simulink model "Inverse_Clark_Park_Transform"  (R2021a)
settings: Solver=FixedStepAuto  StartTime=0.0  StopTime=10  FixedStep=2e-5  RelTol=1e-6
InitFcn:
  | cd 'F:\Learning\Power\FOC';
  | run('Params.m')
settings Model: Creator=DEEL  LastModifiedBy=DEEL
settings SolverCC: ZeroCrossControl=DisableAll
settings DataIOCC: SaveOutput=off  SaveTime=off
settings OptimizationCC: DefaultParameterBehavior=Inlined  EnhancedBackFolding=on  PassReuseOutputArgsAs=Individual arguments  ZeroExternalMemoryAtStartup=off  ZeroInternalMemoryAtStartup=off  OptimizeBlockOrder=speed  DifferentSizesBufferReuse=on  OptimizationCustomize=off  EfficientTunableParamExpr=on
settings DebuggingCC: ParameterTunabilityLossMsg=error
settings SFSimCC: MATLABDynamicMemAlloc=off
settings RTWCC: SystemTargetFile=ert.tlc  TemplateMakefile=ert_default_tmf
settings CodeAppCC: ForceParamTrailComments=on  IgnoreCustomStorageClasses=off  OperatorAnnotations=on  SimulinkDataObjDesc=on  SFDataObjDesc=on  InsertBlockDesc=on
settings ERTTargetCC: TargetLangStandard=C99 (ISO)  GenerateSampleERTMain=on  InlinedParameterPlacement=NonHierarchical  ERTCustomFileTemplate=example_file_process.tlc

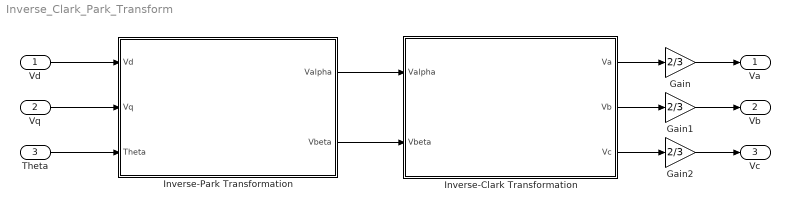
== system Inverse_Clark_Park_Transform ==
  Vd : Inport  OutDataTypeStr=double  PortDimensions=1  SampleTime=0
  Vq : Inport  Port=2  OutDataTypeStr=double  PortDimensions=1  SampleTime=0
  Theta : Inport  Port=3  OutDataTypeStr=double  PortDimensions=1  SampleTime=0
  Gain : Gain  Gain=2/3
  Gain1 : Gain  Gain=2/3
  Gain2 : Gain  Gain=2/3
  Inverse-Clark Transformation : Subsystem
  Inverse-Park Transformation : Subsystem
  Va : Outport  OutDataTypeStr=double  PortDimensions=1  SampleTime=0
  Vb : Outport  Port=2  OutDataTypeStr=double  PortDimensions=1  SampleTime=0
  Vc : Outport  Port=3  OutDataTypeStr=double  PortDimensions=1  SampleTime=0
  wires:
  Inverse-Clark Transformation/2(Vb) -> Gain1/1
  Inverse-Clark Transformation/1(Va) -> Gain/1
  Inverse-Park Transformation/2(Vbeta) -> Inverse-Clark Transformation/2(Vbeta)
  Inverse-Park Transformation/1(Valpha) -> Inverse-Clark Transformation/1(Valpha)
  Gain/1 -> Va/1
  Gain1/1 -> Vb/1
  Gain2/1 -> Vc/1
  Inverse-Clark Transformation/3(Vc) -> Gain2/1
  Vd/1 -> Inverse-Park Transformation/1(Vd)
  Vq/1 -> Inverse-Park Transformation/2(Vq)
  Theta/1 -> Inverse-Park Transformation/3(Theta)

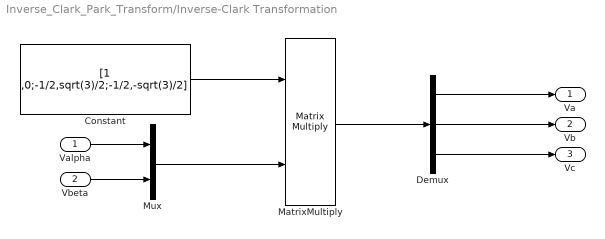
== system Inverse_Clark_Park_Transform/Inverse-Clark Transformation ==
  Valpha : Inport
  Vbeta : Inport  Port=2
  Constant : Constant  Value=[1 ,0;-1/2,sqrt(3)/2;-1/2,-sqrt(3)/2]
  Demux : Demux  Outputs=3
  MatrixMultiply : Product  Multiplication=Matrix(*)
  Mux : Mux  Inputs=2
  Va : Outport
  Vb : Outport  Port=2
  Vc : Outport  Port=3
  wires:
  Demux/3 -> Vc/1
  Valpha/1 -> Mux/1
  Vbeta/1 -> Mux/2
  Constant/1 -> MatrixMultiply/1
  Mux/1 -> MatrixMultiply/2
  MatrixMultiply/1 -> Demux/1
  Demux/1 -> Va/1
  Demux/2 -> Vb/1

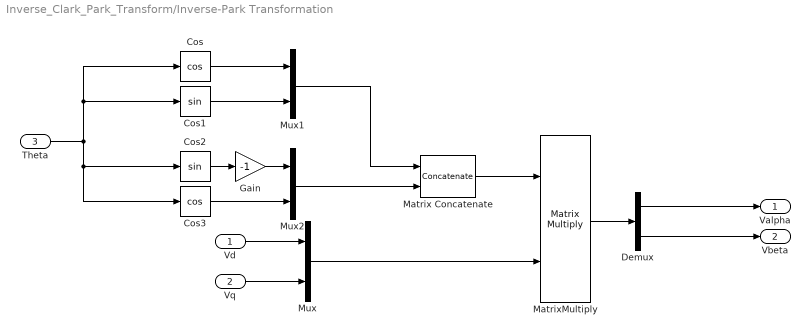
== system Inverse_Clark_Park_Transform/Inverse-Park Transformation ==
  Vd : Inport
  Vq : Inport  Port=2
  Theta : Inport  Port=3
  Cos : Trigonometry  Operator=cos
  Cos1 : Trigonometry
  Cos2 : Trigonometry
  Cos3 : Trigonometry  Operator=cos
  Demux : Demux  Outputs=2
  Gain : Gain  Gain=-1
  Matrix Concatenate : Concatenate  Mode=Multidimensional array  ConcatenateDimension=2
  MatrixMultiply : Product  Multiplication=Matrix(*)
  Mux : Mux  Inputs=2
  Mux1 : Mux  Inputs=2
  Mux2 : Mux  Inputs=2
  Valpha : Outport
  Vbeta : Outport  Port=2
  wires:
  Gain/1 -> Mux2/1
  Matrix Concatenate/1 -> MatrixMultiply/1
  Vq/1 -> Mux/2
  Cos2/1 -> Gain/1
  Theta/1 -> Cos2/1, Cos3/1, Cos1/1, Cos/1
  Mux1/1 -> Matrix Concatenate/1
  Cos/1 -> Mux1/1
  Mux2/1 -> Matrix Concatenate/2
  Cos1/1 -> Mux1/2
  Cos3/1 -> Mux2/2
  Vd/1 -> Mux/1
  Mux/1 -> MatrixMultiply/2
  MatrixMultiply/1 -> Demux/1
  Demux/1 -> Valpha/1
  Demux/2 -> Vbeta/1
